simulink model "RLSS_Functional"  (R2024b)
settings: Solver=VariableStepAuto  StartTime=0.0  StopTime=10.0  RelTol=1e-3
settings Model: Creator=Sadia Dina  LastModifiedBy=Sadia Dina

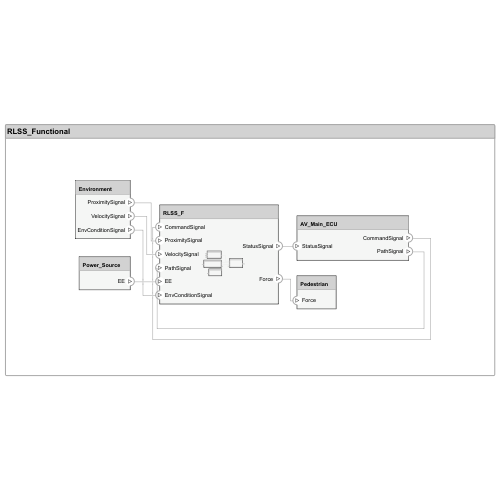
[thumbnail: Simulink's stored preview of the top-level diagram]
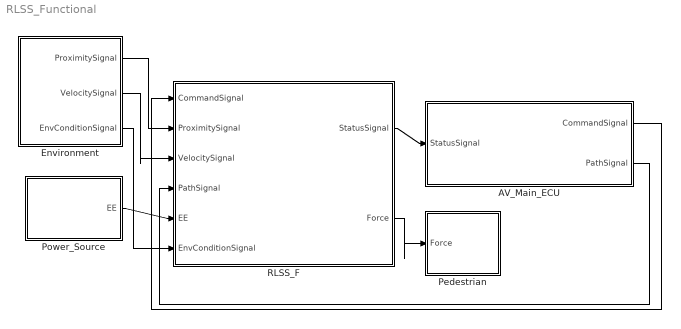
== system RLSS_Functional ==
  AV_Main_ECU : Subsystem
      settings: PortSchema="{\"entries\":[{\"content\":{\"headerSize\":26,\"margin\":15,\"minimumSpacing\":25,\"sides\":[{\"content\":{\"connectorIds\":[\"In1\"]},\"type\":\"ConnectorPlacement.EquallySpacedRectSide\",\"uuid\":\"0e4af77a-90a9-4684-8ac4-a4b6cbc7152a\"},{\"content\":{\"connectorIds\":[\"Out1\",\"Out2\"],\"side\":\"RIGHT\"},\"type\":\"ConnectorPlacement.EquallySpacedRectSide\",\"uuid\":\"aea4d113-8d19-4a11-8a7a-403461391653\"},{\"content\":{\"side\":\"TOP\"},\"type\":\"ConnectorPlacement.EquallySpacedRectSide\",\"uuid\":\"fac91644-aa49-47b2-b805-0dea4a5ff633\"}]},\"type\":\"ConnectorPlacement.EquallySpacedConnector\",\"uuid\":\"0a4b06d2-cdbe-40cc-baaa-fb267f4742e4\"}],\"packageUris\":[\"http://schema.mathworks.com/mf0/Connector/R2020b\"],\"version\":\"1.0\"}"
  Environment : Subsystem
      settings: PortSchema="{\"entries\":[{\"content\":{\"headerSize\":26,\"margin\":15,\"minimumSpacing\":25,\"sides\":[{\"content\":{},\"type\":\"ConnectorPlacement.EquallySpacedRectSide\",\"uuid\":\"0e4af77a-90a9-4684-8ac4-a4b6cbc7152a\"},{\"content\":{\"connectorIds\":[\"Out1\",\"Out2\",\"Out3\"],\"side\":\"RIGHT\"},\"type\":\"ConnectorPlacement.EquallySpacedRectSide\",\"uuid\":\"aea4d113-8d19-4a11-8a7a-403461391653\"},{\"content\":{\"side\":\"TOP\"},\"type\":\"ConnectorPlacement.EquallySpacedRectSide\",\"uuid\":\"fac91644-aa49-47b2-b805-0dea4a5ff633\"}]},\"type\":\"ConnectorPlacement.EquallySpacedConnector\",\"uuid\":\"0a4b06d2-cdbe-40cc-baaa-fb267f4742e4\"}],\"packageUris\":[\"http://schema.mathworks.com/mf0/Connector/R2020b\"],\"version\":\"1.0\"}"
  Pedestrian : Subsystem
      settings: PortSchema="{\"entries\":[{\"content\":{\"headerSize\":26,\"margin\":15,\"minimumSpacing\":25,\"sides\":[{\"content\":{\"connectorIds\":[\"In1\"]},\"type\":\"ConnectorPlacement.EquallySpacedRectSide\",\"uuid\":\"0e4af77a-90a9-4684-8ac4-a4b6cbc7152a\"},{\"content\":{\"side\":\"RIGHT\"},\"type\":\"ConnectorPlacement.EquallySpacedRectSide\",\"uuid\":\"aea4d113-8d19-4a11-8a7a-403461391653\"},{\"content\":{\"side\":\"TOP\"},\"type\":\"ConnectorPlacement.EquallySpacedRectSide\",\"uuid\":\"fac91644-aa49-47b2-b805-0dea4a5ff633\"}]},\"type\":\"ConnectorPlacement.EquallySpacedConnector\",\"uuid\":\"0a4b06d2-cdbe-40cc-baaa-fb267f4742e4\"}],\"packageUris\":[\"http://schema.mathworks.com/mf0/Connector/R2020b\"],\"version\":\"1.0\"}"
  Power_Source : Subsystem
      settings: PortSchema="{\"entries\":[{\"content\":{\"headerSize\":26,\"margin\":15,\"minimumSpacing\":25,\"sides\":[{\"content\":{},\"type\":\"ConnectorPlacement.EquallySpacedRectSide\",\"uuid\":\"0e4af77a-90a9-4684-8ac4-a4b6cbc7152a\"},{\"content\":{\"connectorIds\":[\"Out1\"],\"side\":\"RIGHT\"},\"type\":\"ConnectorPlacement.EquallySpacedRectSide\",\"uuid\":\"aea4d113-8d19-4a11-8a7a-403461391653\"},{\"content\":{\"side\":\"TOP\"},\"type\":\"ConnectorPlacement.EquallySpacedRectSide\",\"uuid\":\"fac91644-aa49-47b2-b805-0dea4a5ff633\"}]},\"type\":\"ConnectorPlacement.EquallySpacedConnector\",\"uuid\":\"0a4b06d2-cdbe-40cc-baaa-fb267f4742e4\"}],\"packageUris\":[\"http://schema.mathworks.com/mf0/Connector/R2020b\"],\"version\":\"1.0\"}"
  RLSS_F : Subsystem
      settings: PortSchema="{\"entries\":[{\"content\":{\"headerSize\":26,\"margin\":15,\"minimumSpacing\":25,\"sides\":[{\"content\":{\"connectorIds\":[\"In1\",\"In2\",\"In3\",\"In4\",\"In5\",\"In6\"]},\"type\":\"ConnectorPlacement.EquallySpacedRectSide\",\"uuid\":\"0e4af77a-90a9-4684-8ac4-a4b6cbc7152a\"},{\"content\":{\"connectorIds\":[\"Out1\",\"Out2\"],\"side\":\"RIGHT\"},\"type\":\"ConnectorPlacement.EquallySpacedRectSide\",\"uuid\":\"aea4d113-8d19-4a11-8a7a-403461391653\"},{\"content\":{\"side\":\"TOP\"},\"type\":\"ConnectorPlacement.EquallySpacedRectSide\",\"uuid\":\"fac91644-aa49-47b2-b805-0dea4a5ff633\"}]},\"type\":\"ConnectorPlacement.EquallySpacedConnector\",\"uuid\":\"0a4b06d2-cdbe-40cc-baaa-fb267f4742e4\"}],\"packageUris\":[\"http://schema.mathworks.com/mf0/Connector/R2020b\"],\"version\":\"1.0\"}"
  wires:
  Environment/1(ProximitySignal) -> RLSS_F/2(ProximitySignal)
  Environment/2(VelocitySignal) -> RLSS_F/3(VelocitySignal)
  Power_Source/1(EE) -> RLSS_F/5(EE)
  Environment/3(EnvConditionSignal) -> RLSS_F/6(EnvConditionSignal)
  RLSS_F/2(Force) -> Pedestrian/1(Force)
  RLSS_F/1(StatusSignal) -> AV_Main_ECU/1(StatusSignal)
  AV_Main_ECU/2(PathSignal) -> RLSS_F/4(PathSignal)
  AV_Main_ECU/1(CommandSignal) -> RLSS_F/1(CommandSignal)

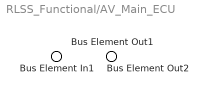
== system RLSS_Functional/AV_Main_ECU ==
  Bus Element In1 : Inport  PortName=StatusSignal
  Bus Element Out1 : Outport  PortName=CommandSignal
  Bus Element Out2 : Outport  Port=2  PortName=PathSignal

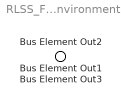
== system RLSS_Functional/Environment ==
  Bus Element Out1 : Outport  PortName=ProximitySignal
  Bus Element Out2 : Outport  Port=2  PortName=VelocitySignal
  Bus Element Out3 : Outport  Port=3  PortName=EnvConditionSignal

== system RLSS_Functional/Pedestrian ==
  Bus Element In1 : Inport  PortName=Force

== system RLSS_Functional/Power_Source ==
  Bus Element Out1 : Outport  PortName=EE

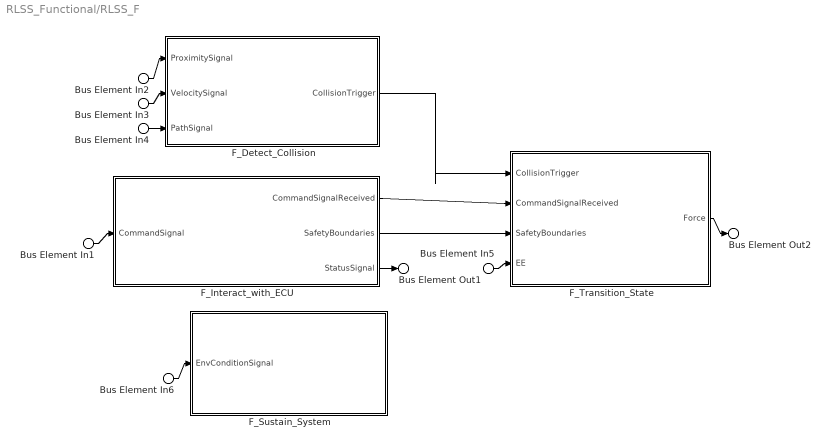
== system RLSS_Functional/RLSS_F ==
  Bus Element In1 : Inport  PortName=CommandSignal
  Bus Element In2 : Inport  Port=2  PortName=ProximitySignal
  Bus Element In3 : Inport  Port=3  PortName=VelocitySignal
  Bus Element In4 : Inport  Port=4  PortName=PathSignal
  Bus Element In5 : Inport  Port=5  PortName=EE
  Bus Element In6 : Inport  Port=6  PortName=EnvConditionSignal
  F_Detect_Collision : Subsystem
      settings: PortSchema="{\"entries\":[{\"content\":{\"headerSize\":26,\"margin\":15,\"minimumSpacing\":25,\"sides\":[{\"content\":{\"connectorIds\":[\"In1\",\"In2\",\"In3\"]},\"type\":\"ConnectorPlacement.EquallySpacedRectSide\",\"uuid\":\"0e4af77a-90a9-4684-8ac4-a4b6cbc7152a\"},{\"content\":{\"connectorIds\":[\"Out1\"],\"side\":\"RIGHT\"},\"type\":\"ConnectorPlacement.EquallySpacedRectSide\",\"uuid\":\"aea4d113-8d19-4a11-8a7a-403461391653\"},{\"content\":{\"side\":\"TOP\"},\"type\":\"ConnectorPlacement.EquallySpacedRectSide\",\"uuid\":\"fac91644-aa49-47b2-b805-0dea4a5ff633\"}]},\"type\":\"ConnectorPlacement.EquallySpacedConnector\",\"uuid\":\"0a4b06d2-cdbe-40cc-baaa-fb267f4742e4\"}],\"packageUris\":[\"http://schema.mathworks.com/mf0/Connector/R2020b\"],\"version\":\"1.0\"}"
  F_Interact_with_ECU : Subsystem
      settings: PortSchema="{\"entries\":[{\"content\":{\"headerSize\":26,\"margin\":15,\"minimumSpacing\":25,\"sides\":[{\"content\":{\"connectorIds\":[\"In1\"]},\"type\":\"ConnectorPlacement.EquallySpacedRectSide\",\"uuid\":\"0e4af77a-90a9-4684-8ac4-a4b6cbc7152a\"},{\"content\":{\"connectorIds\":[\"Out1\",\"Out2\",\"Out3\"],\"side\":\"RIGHT\"},\"type\":\"ConnectorPlacement.EquallySpacedRectSide\",\"uuid\":\"aea4d113-8d19-4a11-8a7a-403461391653\"},{\"content\":{\"side\":\"TOP\"},\"type\":\"ConnectorPlacement.EquallySpacedRectSide\",\"uuid\":\"fac91644-aa49-47b2-b805-0dea4a5ff633\"}]},\"type\":\"ConnectorPlacement.EquallySpacedConnector\",\"uuid\":\"0a4b06d2-cdbe-40cc-baaa-fb267f4742e4\"}],\"packageUris\":[\"http://schema.mathworks.com/mf0/Connector/R2020b\"],\"version\":\"1.0\"}"
  F_Sustain_System : Subsystem
      settings: PortSchema="{\"entries\":[{\"content\":{\"headerSize\":26,\"margin\":15,\"minimumSpacing\":25,\"sides\":[{\"content\":{\"connectorIds\":[\"In1\"]},\"type\":\"ConnectorPlacement.EquallySpacedRectSide\",\"uuid\":\"0e4af77a-90a9-4684-8ac4-a4b6cbc7152a\"},{\"content\":{\"side\":\"RIGHT\"},\"type\":\"ConnectorPlacement.EquallySpacedRectSide\",\"uuid\":\"aea4d113-8d19-4a11-8a7a-403461391653\"},{\"content\":{\"side\":\"TOP\"},\"type\":\"ConnectorPlacement.EquallySpacedRectSide\",\"uuid\":\"fac91644-aa49-47b2-b805-0dea4a5ff633\"}]},\"type\":\"ConnectorPlacement.EquallySpacedConnector\",\"uuid\":\"0a4b06d2-cdbe-40cc-baaa-fb267f4742e4\"}],\"packageUris\":[\"http://schema.mathworks.com/mf0/Connector/R2020b\"],\"version\":\"1.0\"}"
  F_Transition_State : Subsystem
      settings: PortSchema="{\"entries\":[{\"content\":{\"headerSize\":26,\"margin\":15,\"minimumSpacing\":25,\"sides\":[{\"content\":{\"connectorIds\":[\"In1\",\"In2\",\"In3\",\"In4\"]},\"type\":\"ConnectorPlacement.EquallySpacedRectSide\",\"uuid\":\"0e4af77a-90a9-4684-8ac4-a4b6cbc7152a\"},{\"content\":{\"connectorIds\":[\"Out1\"],\"side\":\"RIGHT\"},\"type\":\"ConnectorPlacement.EquallySpacedRectSide\",\"uuid\":\"aea4d113-8d19-4a11-8a7a-403461391653\"},{\"content\":{\"side\":\"TOP\"},\"type\":\"ConnectorPlacement.EquallySpacedRectSide\",\"uuid\":\"fac91644-aa49-47b2-b805-0dea4a5ff633\"}]},\"type\":\"ConnectorPlacement.EquallySpacedConnector\",\"uuid\":\"0a4b06d2-cdbe-40cc-baaa-fb267f4742e4\"}],\"packageUris\":[\"http://schema.mathworks.com/mf0/Connector/R2020b\"],\"version\":\"1.0\"}"
  Bus Element Out1 : Outport  PortName=StatusSignal
  Bus Element Out2 : Outport  Port=2  PortName=Force
  wires:
  F_Detect_Collision/1(CollisionTrigger) -> F_Transition_State/1(CollisionTrigger)
  F_Interact_with_ECU/1(CommandSignalReceived) -> F_Transition_State/2(CommandSignalReceived)
  F_Interact_with_ECU/2(SafetyBoundaries) -> F_Transition_State/3(SafetyBoundaries)
  Bus Element In1/1 -> F_Interact_with_ECU/1(CommandSignal)
  Bus Element In2/1 -> F_Detect_Collision/1(ProximitySignal)
  Bus Element In3/1 -> F_Detect_Collision/2(VelocitySignal)
  Bus Element In4/1 -> F_Detect_Collision/3(PathSignal)
  Bus Element In5/1 -> F_Transition_State/4(EE)
  Bus Element In6/1 -> F_Sustain_System/1(EnvConditionSignal)
  F_Transition_State/1(Force) -> Bus Element Out2/1
  F_Interact_with_ECU/3(StatusSignal) -> Bus Element Out1/1

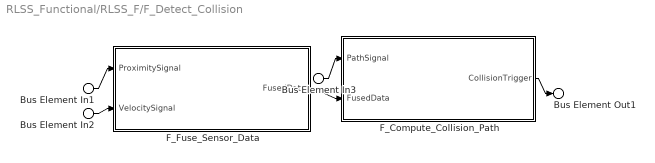
== system RLSS_Functional/RLSS_F/F_Detect_Collision ==
  Bus Element In1 : Inport  PortName=ProximitySignal
  Bus Element In2 : Inport  Port=2  PortName=VelocitySignal
  Bus Element In3 : Inport  Port=3  PortName=PathSignal
  F_Compute_Collision_Path : Subsystem
      settings: PortSchema="{\"entries\":[{\"content\":{\"headerSize\":26,\"margin\":15,\"minimumSpacing\":25,\"sides\":[{\"content\":{\"connectorIds\":[\"In1\",\"In2\"]},\"type\":\"ConnectorPlacement.EquallySpacedRectSide\",\"uuid\":\"0e4af77a-90a9-4684-8ac4-a4b6cbc7152a\"},{\"content\":{\"connectorIds\":[\"Out1\"],\"side\":\"RIGHT\"},\"type\":\"ConnectorPlacement.EquallySpacedRectSide\",\"uuid\":\"aea4d113-8d19-4a11-8a7a-403461391653\"},{\"content\":{\"side\":\"TOP\"},\"type\":\"ConnectorPlacement.EquallySpacedRectSide\",\"uuid\":\"fac91644-aa49-47b2-b805-0dea4a5ff633\"}]},\"type\":\"ConnectorPlacement.EquallySpacedConnector\",\"uuid\":\"0a4b06d2-cdbe-40cc-baaa-fb267f4742e4\"}],\"packageUris\":[\"http://schema.mathworks.com/mf0/Connector/R2020b\"],\"version\":\"1.0\"}"
  F_Fuse_Sensor_Data : Subsystem
      settings: PortSchema="{\"entries\":[{\"content\":{\"headerSize\":26,\"margin\":15,\"minimumSpacing\":25,\"sides\":[{\"content\":{\"connectorIds\":[\"In1\",\"In2\"]},\"type\":\"ConnectorPlacement.EquallySpacedRectSide\",\"uuid\":\"0e4af77a-90a9-4684-8ac4-a4b6cbc7152a\"},{\"content\":{\"connectorIds\":[\"Out1\"],\"side\":\"RIGHT\"},\"type\":\"ConnectorPlacement.EquallySpacedRectSide\",\"uuid\":\"aea4d113-8d19-4a11-8a7a-403461391653\"},{\"content\":{\"side\":\"TOP\"},\"type\":\"ConnectorPlacement.EquallySpacedRectSide\",\"uuid\":\"fac91644-aa49-47b2-b805-0dea4a5ff633\"}]},\"type\":\"ConnectorPlacement.EquallySpacedConnector\",\"uuid\":\"0a4b06d2-cdbe-40cc-baaa-fb267f4742e4\"}],\"packageUris\":[\"http://schema.mathworks.com/mf0/Connector/R2020b\"],\"version\":\"1.0\"}"
  Bus Element Out1 : Outport  PortName=CollisionTrigger
  wires:
  F_Fuse_Sensor_Data/1(FusedData) -> F_Compute_Collision_Path/2(FusedData)
  Bus Element In1/1 -> F_Fuse_Sensor_Data/1(ProximitySignal)
  Bus Element In2/1 -> F_Fuse_Sensor_Data/2(VelocitySignal)
  Bus Element In3/1 -> F_Compute_Collision_Path/1(PathSignal)
  F_Compute_Collision_Path/1(CollisionTrigger) -> Bus Element Out1/1

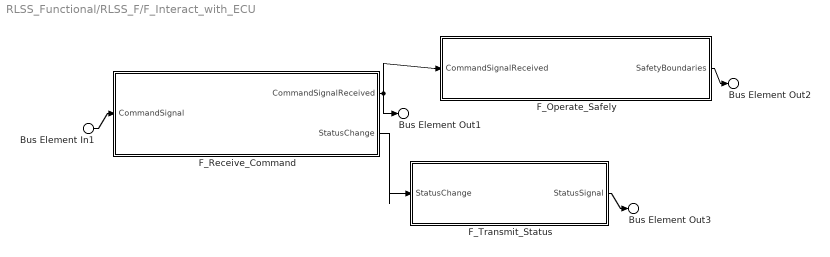
== system RLSS_Functional/RLSS_F/F_Interact_with_ECU ==
  Bus Element In1 : Inport  PortName=CommandSignal
  F_Operate_Safely : Subsystem
      settings: PortSchema="{\"entries\":[{\"content\":{\"headerSize\":26,\"margin\":15,\"minimumSpacing\":25,\"sides\":[{\"content\":{\"connectorIds\":[\"In1\"]},\"type\":\"ConnectorPlacement.EquallySpacedRectSide\",\"uuid\":\"0e4af77a-90a9-4684-8ac4-a4b6cbc7152a\"},{\"content\":{\"connectorIds\":[\"Out1\"],\"side\":\"RIGHT\"},\"type\":\"ConnectorPlacement.EquallySpacedRectSide\",\"uuid\":\"aea4d113-8d19-4a11-8a7a-403461391653\"},{\"content\":{\"side\":\"TOP\"},\"type\":\"ConnectorPlacement.EquallySpacedRectSide\",\"uuid\":\"fac91644-aa49-47b2-b805-0dea4a5ff633\"}]},\"type\":\"ConnectorPlacement.EquallySpacedConnector\",\"uuid\":\"0a4b06d2-cdbe-40cc-baaa-fb267f4742e4\"}],\"packageUris\":[\"http://schema.mathworks.com/mf0/Connector/R2020b\"],\"version\":\"1.0\"}"
  F_Receive_Command : Subsystem
      settings: PortSchema="{\"entries\":[{\"content\":{\"headerSize\":26,\"margin\":15,\"minimumSpacing\":25,\"sides\":[{\"content\":{\"connectorIds\":[\"In1\"]},\"type\":\"ConnectorPlacement.EquallySpacedRectSide\",\"uuid\":\"0e4af77a-90a9-4684-8ac4-a4b6cbc7152a\"},{\"content\":{\"connectorIds\":[\"Out1\",\"Out2\"],\"side\":\"RIGHT\"},\"type\":\"ConnectorPlacement.EquallySpacedRectSide\",\"uuid\":\"aea4d113-8d19-4a11-8a7a-403461391653\"},{\"content\":{\"side\":\"TOP\"},\"type\":\"ConnectorPlacement.EquallySpacedRectSide\",\"uuid\":\"fac91644-aa49-47b2-b805-0dea4a5ff633\"}]},\"type\":\"ConnectorPlacement.EquallySpacedConnector\",\"uuid\":\"0a4b06d2-cdbe-40cc-baaa-fb267f4742e4\"}],\"packageUris\":[\"http://schema.mathworks.com/mf0/Connector/R2020b\"],\"version\":\"1.0\"}"
  F_Transmit_Status : Subsystem
      settings: PortSchema="{\"entries\":[{\"content\":{\"headerSize\":26,\"margin\":15,\"minimumSpacing\":25,\"sides\":[{\"content\":{\"connectorIds\":[\"In1\"]},\"type\":\"ConnectorPlacement.EquallySpacedRectSide\",\"uuid\":\"0e4af77a-90a9-4684-8ac4-a4b6cbc7152a\"},{\"content\":{\"connectorIds\":[\"Out1\"],\"side\":\"RIGHT\"},\"type\":\"ConnectorPlacement.EquallySpacedRectSide\",\"uuid\":\"aea4d113-8d19-4a11-8a7a-403461391653\"},{\"content\":{\"side\":\"TOP\"},\"type\":\"ConnectorPlacement.EquallySpacedRectSide\",\"uuid\":\"fac91644-aa49-47b2-b805-0dea4a5ff633\"}]},\"type\":\"ConnectorPlacement.EquallySpacedConnector\",\"uuid\":\"0a4b06d2-cdbe-40cc-baaa-fb267f4742e4\"}],\"packageUris\":[\"http://schema.mathworks.com/mf0/Connector/R2020b\"],\"version\":\"1.0\"}"
  Bus Element Out1 : Outport  PortName=CommandSignalReceived
  Bus Element Out2 : Outport  Port=2  PortName=SafetyBoundaries
  Bus Element Out3 : Outport  Port=3  PortName=StatusSignal
  wires:
  F_Receive_Command/2(StatusChange) -> F_Transmit_Status/1(StatusChange)
  F_Receive_Command/1(CommandSignalReceived) -> Bus Element Out1/1, F_Operate_Safely/1(CommandSignalReceived)
  Bus Element In1/1 -> F_Receive_Command/1(CommandSignal)
  F_Operate_Safely/1(SafetyBoundaries) -> Bus Element Out2/1
  F_Transmit_Status/1(StatusSignal) -> Bus Element Out3/1

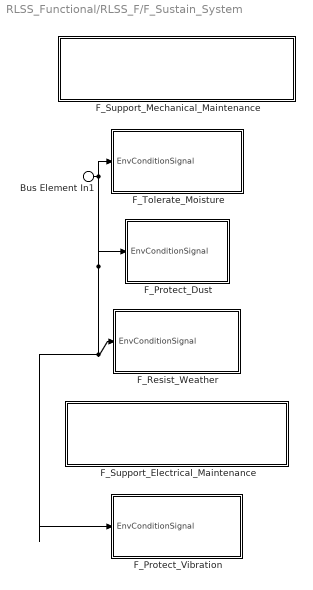
== system RLSS_Functional/RLSS_F/F_Sustain_System ==
  Bus Element In1 : Inport  PortName=EnvConditionSignal
  F_Protect_Dust : Subsystem
      settings: PortSchema="{\"entries\":[{\"content\":{\"headerSize\":26,\"margin\":15,\"minimumSpacing\":25,\"sides\":[{\"content\":{\"connectorIds\":[\"In1\"]},\"type\":\"ConnectorPlacement.EquallySpacedRectSide\",\"uuid\":\"0e4af77a-90a9-4684-8ac4-a4b6cbc7152a\"},{\"content\":{\"side\":\"RIGHT\"},\"type\":\"ConnectorPlacement.EquallySpacedRectSide\",\"uuid\":\"aea4d113-8d19-4a11-8a7a-403461391653\"},{\"content\":{\"side\":\"TOP\"},\"type\":\"ConnectorPlacement.EquallySpacedRectSide\",\"uuid\":\"fac91644-aa49-47b2-b805-0dea4a5ff633\"}]},\"type\":\"ConnectorPlacement.EquallySpacedConnector\",\"uuid\":\"0a4b06d2-cdbe-40cc-baaa-fb267f4742e4\"}],\"packageUris\":[\"http://schema.mathworks.com/mf0/Connector/R2020b\"],\"version\":\"1.0\"}"
  F_Protect_Vibration : Subsystem
      settings: PortSchema="{\"entries\":[{\"content\":{\"headerSize\":26,\"margin\":15,\"minimumSpacing\":25,\"sides\":[{\"content\":{\"connectorIds\":[\"In1\"]},\"type\":\"ConnectorPlacement.EquallySpacedRectSide\",\"uuid\":\"0e4af77a-90a9-4684-8ac4-a4b6cbc7152a\"},{\"content\":{\"side\":\"RIGHT\"},\"type\":\"ConnectorPlacement.EquallySpacedRectSide\",\"uuid\":\"aea4d113-8d19-4a11-8a7a-403461391653\"},{\"content\":{\"side\":\"TOP\"},\"type\":\"ConnectorPlacement.EquallySpacedRectSide\",\"uuid\":\"fac91644-aa49-47b2-b805-0dea4a5ff633\"}]},\"type\":\"ConnectorPlacement.EquallySpacedConnector\",\"uuid\":\"0a4b06d2-cdbe-40cc-baaa-fb267f4742e4\"}],\"packageUris\":[\"http://schema.mathworks.com/mf0/Connector/R2020b\"],\"version\":\"1.0\"}"
  F_Resist_Weather : Subsystem
      settings: PortSchema="{\"entries\":[{\"content\":{\"headerSize\":26,\"margin\":15,\"minimumSpacing\":25,\"sides\":[{\"content\":{\"connectorIds\":[\"In1\"]},\"type\":\"ConnectorPlacement.EquallySpacedRectSide\",\"uuid\":\"0e4af77a-90a9-4684-8ac4-a4b6cbc7152a\"},{\"content\":{\"side\":\"RIGHT\"},\"type\":\"ConnectorPlacement.EquallySpacedRectSide\",\"uuid\":\"aea4d113-8d19-4a11-8a7a-403461391653\"},{\"content\":{\"side\":\"TOP\"},\"type\":\"ConnectorPlacement.EquallySpacedRectSide\",\"uuid\":\"fac91644-aa49-47b2-b805-0dea4a5ff633\"}]},\"type\":\"ConnectorPlacement.EquallySpacedConnector\",\"uuid\":\"0a4b06d2-cdbe-40cc-baaa-fb267f4742e4\"}],\"packageUris\":[\"http://schema.mathworks.com/mf0/Connector/R2020b\"],\"version\":\"1.0\"}"
  F_Support_Electrical_Maintenance : Subsystem
      settings: PortSchema="{\"entries\":[{\"content\":{\"headerSize\":26,\"margin\":15,\"minimumSpacing\":25,\"sides\":[{\"content\":{},\"type\":\"ConnectorPlacement.EquallySpacedRectSide\",\"uuid\":\"0e4af77a-90a9-4684-8ac4-a4b6cbc7152a\"},{\"content\":{\"side\":\"RIGHT\"},\"type\":\"ConnectorPlacement.EquallySpacedRectSide\",\"uuid\":\"aea4d113-8d19-4a11-8a7a-403461391653\"},{\"content\":{\"side\":\"TOP\"},\"type\":\"ConnectorPlacement.EquallySpacedRectSide\",\"uuid\":\"fac91644-aa49-47b2-b805-0dea4a5ff633\"}]},\"type\":\"ConnectorPlacement.EquallySpacedConnector\",\"uuid\":\"0a4b06d2-cdbe-40cc-baaa-fb267f4742e4\"}],\"packageUris\":[\"http://schema.mathworks.com/mf0/Connector/R2020b\"],\"version\":\"1.0\"}"
  F_Support_Mechanical_Maintenance : Subsystem
      settings: PortSchema="{\"entries\":[{\"content\":{\"headerSize\":26,\"margin\":15,\"minimumSpacing\":25,\"sides\":[{\"content\":{},\"type\":\"ConnectorPlacement.EquallySpacedRectSide\",\"uuid\":\"0e4af77a-90a9-4684-8ac4-a4b6cbc7152a\"},{\"content\":{\"side\":\"RIGHT\"},\"type\":\"ConnectorPlacement.EquallySpacedRectSide\",\"uuid\":\"aea4d113-8d19-4a11-8a7a-403461391653\"},{\"content\":{\"side\":\"TOP\"},\"type\":\"ConnectorPlacement.EquallySpacedRectSide\",\"uuid\":\"fac91644-aa49-47b2-b805-0dea4a5ff633\"}]},\"type\":\"ConnectorPlacement.EquallySpacedConnector\",\"uuid\":\"0a4b06d2-cdbe-40cc-baaa-fb267f4742e4\"}],\"packageUris\":[\"http://schema.mathworks.com/mf0/Connector/R2020b\"],\"version\":\"1.0\"}"
  F_Tolerate_Moisture : Subsystem
      settings: PortSchema="{\"entries\":[{\"content\":{\"headerSize\":26,\"margin\":15,\"minimumSpacing\":25,\"sides\":[{\"content\":{\"connectorIds\":[\"In1\"]},\"type\":\"ConnectorPlacement.EquallySpacedRectSide\",\"uuid\":\"0e4af77a-90a9-4684-8ac4-a4b6cbc7152a\"},{\"content\":{\"side\":\"RIGHT\"},\"type\":\"ConnectorPlacement.EquallySpacedRectSide\",\"uuid\":\"aea4d113-8d19-4a11-8a7a-403461391653\"},{\"content\":{\"side\":\"TOP\"},\"type\":\"ConnectorPlacement.EquallySpacedRectSide\",\"uuid\":\"fac91644-aa49-47b2-b805-0dea4a5ff633\"}]},\"type\":\"ConnectorPlacement.EquallySpacedConnector\",\"uuid\":\"0a4b06d2-cdbe-40cc-baaa-fb267f4742e4\"}],\"packageUris\":[\"http://schema.mathworks.com/mf0/Connector/R2020b\"],\"version\":\"1.0\"}"
  wires:
  Bus Element In1/1 -> F_Protect_Vibration/1(EnvConditionSignal), F_Resist_Weather/1(EnvConditionSignal), F_Protect_Dust/1(EnvConditionSignal), F_Tolerate_Moisture/1(EnvConditionSignal)

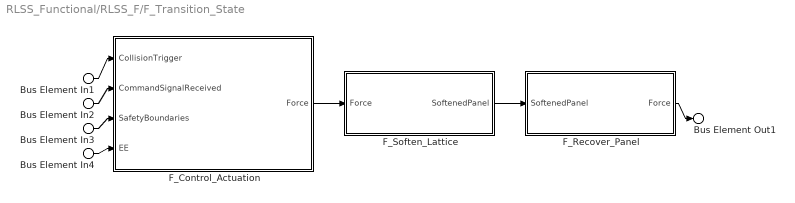
== system RLSS_Functional/RLSS_F/F_Transition_State ==
  Bus Element In1 : Inport  PortName=CollisionTrigger
  Bus Element In2 : Inport  Port=2  PortName=CommandSignalReceived
  Bus Element In3 : Inport  Port=3  PortName=SafetyBoundaries
  Bus Element In4 : Inport  Port=4  PortName=EE
  F_Control_Actuation : Subsystem
      settings: PortSchema="{\"entries\":[{\"content\":{\"headerSize\":26,\"margin\":15,\"minimumSpacing\":25,\"sides\":[{\"content\":{\"connectorIds\":[\"In1\",\"In2\",\"In3\",\"In4\"]},\"type\":\"ConnectorPlacement.EquallySpacedRectSide\",\"uuid\":\"0e4af77a-90a9-4684-8ac4-a4b6cbc7152a\"},{\"content\":{\"connectorIds\":[\"Out1\"],\"side\":\"RIGHT\"},\"type\":\"ConnectorPlacement.EquallySpacedRectSide\",\"uuid\":\"aea4d113-8d19-4a11-8a7a-403461391653\"},{\"content\":{\"side\":\"TOP\"},\"type\":\"ConnectorPlacement.EquallySpacedRectSide\",\"uuid\":\"fac91644-aa49-47b2-b805-0dea4a5ff633\"}]},\"type\":\"ConnectorPlacement.EquallySpacedConnector\",\"uuid\":\"0a4b06d2-cdbe-40cc-baaa-fb267f4742e4\"}],\"packageUris\":[\"http://schema.mathworks.com/mf0/Connector/R2020b\"],\"version\":\"1.0\"}"
  F_Recover_Panel : Subsystem
      settings: PortSchema="{\"entries\":[{\"content\":{\"headerSize\":26,\"margin\":15,\"minimumSpacing\":25,\"sides\":[{\"content\":{\"connectorIds\":[\"In1\"]},\"type\":\"ConnectorPlacement.EquallySpacedRectSide\",\"uuid\":\"0e4af77a-90a9-4684-8ac4-a4b6cbc7152a\"},{\"content\":{\"connectorIds\":[\"Out1\"],\"side\":\"RIGHT\"},\"type\":\"ConnectorPlacement.EquallySpacedRectSide\",\"uuid\":\"aea4d113-8d19-4a11-8a7a-403461391653\"},{\"content\":{\"side\":\"TOP\"},\"type\":\"ConnectorPlacement.EquallySpacedRectSide\",\"uuid\":\"fac91644-aa49-47b2-b805-0dea4a5ff633\"}]},\"type\":\"ConnectorPlacement.EquallySpacedConnector\",\"uuid\":\"0a4b06d2-cdbe-40cc-baaa-fb267f4742e4\"}],\"packageUris\":[\"http://schema.mathworks.com/mf0/Connector/R2020b\"],\"version\":\"1.0\"}"
  F_Soften_Lattice : Subsystem
      settings: PortSchema="{\"entries\":[{\"content\":{\"headerSize\":26,\"margin\":15,\"minimumSpacing\":25,\"sides\":[{\"content\":{\"connectorIds\":[\"In1\"]},\"type\":\"ConnectorPlacement.EquallySpacedRectSide\",\"uuid\":\"0e4af77a-90a9-4684-8ac4-a4b6cbc7152a\"},{\"content\":{\"connectorIds\":[\"Out1\"],\"side\":\"RIGHT\"},\"type\":\"ConnectorPlacement.EquallySpacedRectSide\",\"uuid\":\"aea4d113-8d19-4a11-8a7a-403461391653\"},{\"content\":{\"side\":\"TOP\"},\"type\":\"ConnectorPlacement.EquallySpacedRectSide\",\"uuid\":\"fac91644-aa49-47b2-b805-0dea4a5ff633\"}]},\"type\":\"ConnectorPlacement.EquallySpacedConnector\",\"uuid\":\"0a4b06d2-cdbe-40cc-baaa-fb267f4742e4\"}],\"packageUris\":[\"http://schema.mathworks.com/mf0/Connector/R2020b\"],\"version\":\"1.0\"}"
  Bus Element Out1 : Outport  PortName=Force
  wires:
  F_Soften_Lattice/1(SoftenedPanel) -> F_Recover_Panel/1(SoftenedPanel)
  F_Control_Actuation/1(Force) -> F_Soften_Lattice/1(Force)
  Bus Element In1/1 -> F_Control_Actuation/1(CollisionTrigger)
  Bus Element In2/1 -> F_Control_Actuation/2(CommandSignalReceived)
  Bus Element In3/1 -> F_Control_Actuation/3(SafetyBoundaries)
  Bus Element In4/1 -> F_Control_Actuation/4(EE)
  F_Recover_Panel/1(Force) -> Bus Element Out1/1

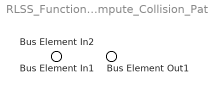
== system RLSS_Functional/RLSS_F/F_Detect_Collision/F_Compute_Collision_Path ==
  Bus Element In1 : Inport  PortName=PathSignal
  Bus Element In2 : Inport  Port=2  PortName=FusedData
  Bus Element Out1 : Outport  PortName=CollisionTrigger

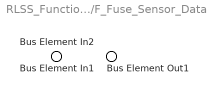
== system RLSS_Functional/RLSS_F/F_Detect_Collision/F_Fuse_Sensor_Data ==
  Bus Element In1 : Inport  PortName=ProximitySignal
  Bus Element In2 : Inport  Port=2  PortName=VelocitySignal
  Bus Element Out1 : Outport  PortName=FusedData

== system RLSS_Functional/RLSS_F/F_Interact_with_ECU/F_Operate_Safely ==
  Bus Element In1 : Inport  PortName=CommandSignalReceived
  Bus Element Out1 : Outport  PortName=SafetyBoundaries

== system RLSS_Functional/RLSS_F/F_Interact_with_ECU/F_Receive_Command ==
  Bus Element In1 : Inport  PortName=CommandSignal
  Bus Element Out1 : Outport  PortName=CommandSignalReceived
  Bus Element Out2 : Outport  Port=2  PortName=StatusChange

== system RLSS_Functional/RLSS_F/F_Interact_with_ECU/F_Transmit_Status ==
  Bus Element In1 : Inport  PortName=StatusChange
  Bus Element Out1 : Outport  PortName=StatusSignal

== system RLSS_Functional/RLSS_F/F_Sustain_System/F_Protect_Dust ==
  Bus Element In1 : Inport  PortName=EnvConditionSignal

== system RLSS_Functional/RLSS_F/F_Sustain_System/F_Protect_Vibration ==
  Bus Element In1 : Inport  PortName=EnvConditionSignal

== system RLSS_Functional/RLSS_F/F_Sustain_System/F_Resist_Weather ==
  Bus Element In1 : Inport  PortName=EnvConditionSignal

== system RLSS_Functional/RLSS_F/F_Sustain_System/F_Support_Electrical_Maintenance ==

== system RLSS_Functional/RLSS_F/F_Sustain_System/F_Support_Mechanical_Maintenance ==

== system RLSS_Functional/RLSS_F/F_Sustain_System/F_Tolerate_Moisture ==
  Bus Element In1 : Inport  PortName=EnvConditionSignal

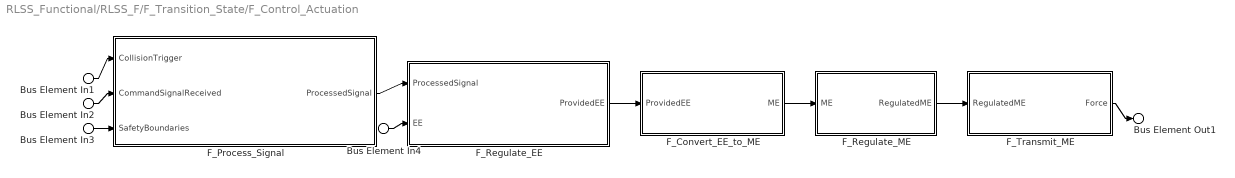
== system RLSS_Functional/RLSS_F/F_Transition_State/F_Control_Actuation ==
  Bus Element In1 : Inport  PortName=CollisionTrigger
  Bus Element In2 : Inport  Port=2  PortName=CommandSignalReceived
  Bus Element In3 : Inport  Port=3  PortName=SafetyBoundaries
  Bus Element In4 : Inport  Port=4  PortName=EE
  F_Convert_EE_to_ME : Subsystem
      settings: PortSchema="{\"entries\":[{\"content\":{\"headerSize\":26,\"margin\":15,\"minimumSpacing\":25,\"sides\":[{\"content\":{\"connectorIds\":[\"In1\"]},\"type\":\"ConnectorPlacement.EquallySpacedRectSide\",\"uuid\":\"0e4af77a-90a9-4684-8ac4-a4b6cbc7152a\"},{\"content\":{\"connectorIds\":[\"Out1\"],\"side\":\"RIGHT\"},\"type\":\"ConnectorPlacement.EquallySpacedRectSide\",\"uuid\":\"aea4d113-8d19-4a11-8a7a-403461391653\"},{\"content\":{\"side\":\"TOP\"},\"type\":\"ConnectorPlacement.EquallySpacedRectSide\",\"uuid\":\"fac91644-aa49-47b2-b805-0dea4a5ff633\"}]},\"type\":\"ConnectorPlacement.EquallySpacedConnector\",\"uuid\":\"0a4b06d2-cdbe-40cc-baaa-fb267f4742e4\"}],\"packageUris\":[\"http://schema.mathworks.com/mf0/Connector/R2020b\"],\"version\":\"1.0\"}"
  F_Process_Signal : Subsystem
      settings: PortSchema="{\"entries\":[{\"content\":{\"headerSize\":26,\"margin\":15,\"minimumSpacing\":25,\"sides\":[{\"content\":{\"connectorIds\":[\"In1\",\"In2\",\"In3\"]},\"type\":\"ConnectorPlacement.EquallySpacedRectSide\",\"uuid\":\"0e4af77a-90a9-4684-8ac4-a4b6cbc7152a\"},{\"content\":{\"connectorIds\":[\"Out1\"],\"side\":\"RIGHT\"},\"type\":\"ConnectorPlacement.EquallySpacedRectSide\",\"uuid\":\"aea4d113-8d19-4a11-8a7a-403461391653\"},{\"content\":{\"side\":\"TOP\"},\"type\":\"ConnectorPlacement.EquallySpacedRectSide\",\"uuid\":\"fac91644-aa49-47b2-b805-0dea4a5ff633\"}]},\"type\":\"ConnectorPlacement.EquallySpacedConnector\",\"uuid\":\"0a4b06d2-cdbe-40cc-baaa-fb267f4742e4\"}],\"packageUris\":[\"http://schema.mathworks.com/mf0/Connector/R2020b\"],\"version\":\"1.0\"}"
  F_Regulate_EE : Subsystem
      settings: PortSchema="{\"entries\":[{\"content\":{\"headerSize\":26,\"margin\":15,\"minimumSpacing\":25,\"sides\":[{\"content\":{\"connectorIds\":[\"In1\",\"In2\"]},\"type\":\"ConnectorPlacement.EquallySpacedRectSide\",\"uuid\":\"0e4af77a-90a9-4684-8ac4-a4b6cbc7152a\"},{\"content\":{\"connectorIds\":[\"Out1\"],\"side\":\"RIGHT\"},\"type\":\"ConnectorPlacement.EquallySpacedRectSide\",\"uuid\":\"aea4d113-8d19-4a11-8a7a-403461391653\"},{\"content\":{\"side\":\"TOP\"},\"type\":\"ConnectorPlacement.EquallySpacedRectSide\",\"uuid\":\"fac91644-aa49-47b2-b805-0dea4a5ff633\"}]},\"type\":\"ConnectorPlacement.EquallySpacedConnector\",\"uuid\":\"0a4b06d2-cdbe-40cc-baaa-fb267f4742e4\"}],\"packageUris\":[\"http://schema.mathworks.com/mf0/Connector/R2020b\"],\"version\":\"1.0\"}"
  F_Regulate_ME : Subsystem
      settings: PortSchema="{\"entries\":[{\"content\":{\"headerSize\":26,\"margin\":15,\"minimumSpacing\":25,\"sides\":[{\"content\":{\"connectorIds\":[\"In1\"]},\"type\":\"ConnectorPlacement.EquallySpacedRectSide\",\"uuid\":\"0e4af77a-90a9-4684-8ac4-a4b6cbc7152a\"},{\"content\":{\"connectorIds\":[\"Out1\"],\"side\":\"RIGHT\"},\"type\":\"ConnectorPlacement.EquallySpacedRectSide\",\"uuid\":\"aea4d113-8d19-4a11-8a7a-403461391653\"},{\"content\":{\"side\":\"TOP\"},\"type\":\"ConnectorPlacement.EquallySpacedRectSide\",\"uuid\":\"fac91644-aa49-47b2-b805-0dea4a5ff633\"}]},\"type\":\"ConnectorPlacement.EquallySpacedConnector\",\"uuid\":\"0a4b06d2-cdbe-40cc-baaa-fb267f4742e4\"}],\"packageUris\":[\"http://schema.mathworks.com/mf0/Connector/R2020b\"],\"version\":\"1.0\"}"
  F_Transmit_ME : Subsystem
      settings: PortSchema="{\"entries\":[{\"content\":{\"headerSize\":26,\"margin\":15,\"minimumSpacing\":25,\"sides\":[{\"content\":{\"connectorIds\":[\"In1\"]},\"type\":\"ConnectorPlacement.EquallySpacedRectSide\",\"uuid\":\"0e4af77a-90a9-4684-8ac4-a4b6cbc7152a\"},{\"content\":{\"connectorIds\":[\"Out1\"],\"side\":\"RIGHT\"},\"type\":\"ConnectorPlacement.EquallySpacedRectSide\",\"uuid\":\"aea4d113-8d19-4a11-8a7a-403461391653\"},{\"content\":{\"side\":\"TOP\"},\"type\":\"ConnectorPlacement.EquallySpacedRectSide\",\"uuid\":\"fac91644-aa49-47b2-b805-0dea4a5ff633\"}]},\"type\":\"ConnectorPlacement.EquallySpacedConnector\",\"uuid\":\"0a4b06d2-cdbe-40cc-baaa-fb267f4742e4\"}],\"packageUris\":[\"http://schema.mathworks.com/mf0/Connector/R2020b\"],\"version\":\"1.0\"}"
  Bus Element Out1 : Outport  PortName=Force
  wires:
  F_Convert_EE_to_ME/1(ME) -> F_Regulate_ME/1(ME)
  F_Regulate_EE/1(ProvidedEE) -> F_Convert_EE_to_ME/1(ProvidedEE)
  F_Process_Signal/1(ProcessedSignal) -> F_Regulate_EE/1(ProcessedSignal)
  F_Regulate_ME/1(RegulatedME) -> F_Transmit_ME/1(RegulatedME)
  Bus Element In1/1 -> F_Process_Signal/1(CollisionTrigger)
  Bus Element In2/1 -> F_Process_Signal/2(CommandSignalReceived)
  Bus Element In3/1 -> F_Process_Signal/3(SafetyBoundaries)
  Bus Element In4/1 -> F_Regulate_EE/2(EE)
  F_Transmit_ME/1(Force) -> Bus Element Out1/1

== system RLSS_Functional/RLSS_F/F_Transition_State/F_Recover_Panel ==
  Bus Element In1 : Inport  PortName=SoftenedPanel
  Bus Element Out1 : Outport  PortName=Force

== system RLSS_Functional/RLSS_F/F_Transition_State/F_Soften_Lattice ==
  Bus Element In1 : Inport  PortName=Force
  Bus Element Out1 : Outport  PortName=SoftenedPanel

== system RLSS_Functional/RLSS_F/F_Transition_State/F_Control_Actuation/F_Convert_EE_to_ME ==
  Bus Element In1 : Inport  PortName=ProvidedEE
  Bus Element Out1 : Outport  PortName=ME

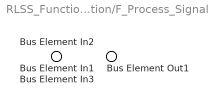
== system RLSS_Functional/RLSS_F/F_Transition_State/F_Control_Actuation/F_Process_Signal ==
  Bus Element In1 : Inport  PortName=CollisionTrigger
  Bus Element In2 : Inport  Port=2  PortName=CommandSignalReceived
  Bus Element In3 : Inport  Port=3  PortName=SafetyBoundaries
  Bus Element Out1 : Outport  PortName=ProcessedSignal

== system RLSS_Functional/RLSS_F/F_Transition_State/F_Control_Actuation/F_Regulate_EE ==
  Bus Element In1 : Inport  PortName=ProcessedSignal
  Bus Element In2 : Inport  Port=2  PortName=EE
  Bus Element Out1 : Outport  PortName=ProvidedEE

== system RLSS_Functional/RLSS_F/F_Transition_State/F_Control_Actuation/F_Regulate_ME ==
  Bus Element In1 : Inport  PortName=ME
  Bus Element Out1 : Outport  PortName=RegulatedME

== system RLSS_Functional/RLSS_F/F_Transition_State/F_Control_Actuation/F_Transmit_ME ==
  Bus Element In1 : Inport  PortName=RegulatedME
  Bus Element Out1 : Outport  PortName=Force
